simulink model "Tractor_HIT_Discrete"  (R2024a)
settings: Solver=ode1  StartTime=0.0  StopTime=60  FixedStep=0.001  RelTol=1e-3
values from neighbouring files (symbols this model uses):
  ANRtarget = 1.05    [Engine1204.sldd]    (also in Engine1204_init_r1.m; Engine2004.sldd; Engine2004_init.m; Engine3204.sldd)
  BackPrs = 3.0 4.2 5.5 7.0 8.5 10.0 11.5 12.5    [Engine1204.sldd]    (also in Engine1204_init_r1.m = [3.0, 4.2, 5.5, 7.0, 8.5, 10.0, 11.5, 12.5]; Engine2004.sldd = 3.0 4.2 5.5 7.0 8.5 10.0 11.5 12.5 13.5 14.5 15.0 15.5 16.0 ; Engine2004_init.m = [3.0,4.2,5.5,7.0,8.5,10.0,11.5,12.5,13.5,14.5,15.0,15.5,16.0; Engine3204.sldd = 3.0 4.5 6.0 7.5 9.0 10.5 12.0 13.0 13.8 14.4 14.8 15.2 15.6 )
  BackPrs_x = 50.0 100.0 150.0 200.0 250.0 300.0 350.0 400.0    [Engine1204.sldd]    (also in Engine1204_init_r1.m = [50:50:400]; Engine2004.sldd = 50.0 100.0 150.0 200.0 250.0 300.0 350.0 400.0 450.0 500.0 5; Engine2004_init.m = [50:50:800]; Engine3204.sldd = 100.0 200.0 300.0 400.0 500.0 600.0 700.0 800.0 900.0 1000.0)
  Bf = 0.38    [Engine1204.sldd]    (also in Engine2004.sldd; Engine3204.sldd)
  Br = 0.47    [Engine1204.sldd]    (also in Engine2004.sldd; Engine3204.sldd)
  BSFC = 320.0 285.0 275.0 280.0 290.0 300.0 310.0 260.0 225.0 215.0 220.0 228.0 240.0 250.0 235.0 208.0 202.0 205.0 212.0 222.0 232.0 230.0 205.0 200.0 204.0 210.0 220.0 230.0 232.0 207.0 203.0 206.0 213.0 224.0 235.0    [Engine1204.sldd]    (also in Engine1204_init_r1.m = [320,285,275,280,290,300,310; Engine2004.sldd = 315.0 280.0 270.0 275.0 285.0 295.0 305.0 255.0 220.0 210.0 ; Engine2004_init.m = [315,280,270,275,285,295,305; Engine3204.sldd = 310.0 275.0 265.0 270.0 280.0 290.0 300.0 250.0 215.0 205.0 )
  BSFC_x = 700.0 1200.0 1400.0 1600.0 1800.0 2000.0 2200.0    [Engine1204.sldd]    (also in Engine1204_init_r1.m = [700,1200,1400,1600,1800,2000,2200]; Engine2004.sldd = 800.0 1200.0 1400.0 1600.0 1800.0 2000.0 2200.0; Engine2004_init.m = [800,1200,1400,1600,1800,2000,2200]; Engine3204.sldd = 800.0 1000.0 1200.0 1400.0 1600.0 1800.0 2100.0)
  BSFC_y = 12.0 24.0 36.0 48.0 54.0    [Engine1204.sldd]    (also in Engine1204_init_r1.m = [12,24,36,48,54]; Engine2004.sldd = 20.0 40.0 60.0 80.0 100.0; Engine2004_init.m = [20,40,60,80,100]; Engine3204.sldd = 30.0 60.0 90.0 120.0 150.0)
  CO = 2.4 1.7 1.5 1.6 1.8 2.1 2.7 1.1 0.72 0.65 0.68 0.78 0.92 1.3 0.7 0.55 0.5 0.53 0.6 0.72 0.95 1.2 0.9 0.85 0.88 0.96 1.1 1.45 3.2 2.3 2.1 2.25 2.5 2.85 3.8    [Engine1204.sldd]    (also in Engine1204_init_r1.m = [; Engine2004.sldd = 2.3 1.63 1.44 1.54 1.73 2.02 2.56 1.05 0.68 0.61 0.64 0.74 0; Engine2004_init.m = [; Engine3204.sldd = 2.2 1.56 1.38 1.48 1.66 1.94 2.46 1.0 0.65 0.58 0.61 0.7 0.8)
  CO_x = 700.0 1200.0 1400.0 1600.0 1800.0 2000.0 2200.0    [Engine1204.sldd]    (also in Engine1204_init_r1.m = [700,1200,1400,1600,1800,2000,2200]; Engine2004.sldd = 800.0 1200.0 1400.0 1600.0 1800.0 2000.0 2200.0; Engine2004_init.m = [800,1200,1400,1600,1800,2000,2200]; Engine3204.sldd = 800.0 1000.0 1200.0 1400.0 1600.0 1800.0 2100.0)
  CO_y = 12.0 24.0 36.0 48.0 54.0    [Engine1204.sldd]    (also in Engine1204_init_r1.m = [12,24,36,48,54]; Engine2004.sldd = 20.0 40.0 60.0 80.0 100.0; Engine2004_init.m = [20,40,60,80,100]; Engine3204.sldd = 30.0 60.0 90.0 120.0 150.0)
  Df = 1.4    [Engine1204.sldd]    (also in Engine2004.sldd; Engine3204.sldd)
  dfmax = 0.1    [Engine1204.sldd]    (also in Engine2004.sldd; Engine3204.sldd)
  dfmin = 0.035    [Engine1204.sldd]    (also in Engine2004.sldd; Engine3204.sldd)
  DOCdPrs = 0.2 0.5 0.8 1.1 1.2    [Engine1204.sldd]    (also in Engine1204_init_r1.m = [0.2  0.5  0.8  1.1  1.2]; Engine2004.sldd = 0.25 0.55 0.85 1.15 1.3; Engine2004_init.m = [0.25,0.55,0.85,1.15,1.30]; Engine3204.sldd = 0.25 0.55 0.85 1.15 1.3 1.45)
  DOCdPrs_x = 50.0 150.0 250.0 350.0 400.0    [Engine1204.sldd]    (also in Engine1204_init_r1.m = [50  150  250  350  400]; Engine2004.sldd = 100.0 250.0 400.0 600.0 800.0; Engine2004_init.m = [100 250 400 600 800]; Engine3204.sldd = 100.0 250.0 400.0 600.0 800.0 1200.0)
  DPFdPrs = 0.3 0.5 0.7 0.9 0.6 1.0 1.4 1.8 0.9 1.5 2.1 2.6 1.2 2.0 2.7 2.8    [Engine1204.sldd]    (also in Engine1204_init_r1.m = [0.3  0.5  0.7  0.9; Engine2004.sldd = 0.35 0.6 0.85 1.1 0.7 1.15 1.6 2.0 1.05 1.7 2.3 2.5 1.4 2.2 ; Engine2004_init.m = [0.35,0.60,0.85,1.10; Engine3204.sldd = 0.35 0.7 1.05 1.4 1.7 2.0 2.2 2.4 2.55 2.65 2.7 2.75 0.6 1.1)
  DPFdPrs_x = 100.0 200.0 300.0 400.0    [Engine1204.sldd]    (also in Engine1204_init_r1.m = [100: 100 : 400]; Engine2004.sldd = 100.0 300.0 500.0 700.0; Engine2004_init.m = [100:200:700]; Engine3204.sldd = 100.0 200.0 300.0 400.0 500.0 600.0 700.0 800.0 900.0 1000.0)
  DPFdPrs_y = 0.0 6.0 12.0 20.0    [Engine1204.sldd]    (also in Engine1204_init_r1.m = [0 6 12 20 ]; Engine2004.sldd = 0.0 8.0 16.0 24.0; Engine2004_init.m = [0 8 16 24]; Engine3204.sldd = 0.0 10.0 20.0 30.0)
  DPFSootBurn = 0.0 0.0 0.0 0.0 0.0 0.2 0.4 0.6 0.8 1.0 1.2 2.4 3.6 4.8 6.0 6.0 12.0 18.0 24.0 30.0 12.0 24.0 36.0 48.0 60.0 20.0 40.0 60.0 80.0 100.0 22.0 44.0 66.0 88.0 110.0    [Engine1204.sldd]    (also in Engine1204_init_r1.m = [0,0,0,0,0; Engine2004.sldd = 0.0 0.0 0.0 0.0 0.0 0.5 1.0 1.5 2.0 2.5 3.0 6.0 9.0 12.0 15.; Engine2004_init.m = [0,0,0,0,0; Engine3204.sldd = 0.0 0.0 0.0 0.0 0.0 0.5 1.0 1.5 2.0 2.5 3.0 6.0 9.0 12.0 15.)
  DPFSootBurn_x = 100.0 200.0 300.0 400.0 500.0    [Engine1204.sldd]    (also in Engine1204_init_r1.m = [100,200,300,400,500]; Engine2004.sldd = 200.0 300.0 400.0 500.0 650.0; Engine2004_init.m = [200,300,400,500,650]; Engine3204.sldd = 200.0 300.0 400.0 500.0 650.0)
  DPFSootBurn_y = 400.0 450.0 500.0 550.0 600.0 650.0 680.0    [Engine1204.sldd]    (also in Engine1204_init_r1.m = [400,450,500,550,600,650,680]; Engine2004.sldd; Engine2004_init.m = [400,450,500,550,600,650,680]; Engine3204.sldd)
  Dr = 1.8    [Engine1204.sldd]    (also in Engine2004.sldd; Engine3204.sldd)
  drmax = 0.12    [Engine1204.sldd]    (also in Engine2004.sldd; Engine3204.sldd)
  drmin = 0.04    [Engine1204.sldd]    (also in Engine2004.sldd; Engine3204.sldd)
  EGRKi = 0.03    [Engine1204.sldd]    (also in Engine1204_init_r1.m; Engine2004.sldd; Engine2004_init.m; Engine3204.sldd)
  EGRKp = 3.5999999999999996    [Engine1204.sldd]    (also in Engine1204_init_r1.m = 3.6; Engine2004.sldd; Engine2004_init.m = 3.6; Engine3204.sldd)
  EGRMax = 1.0    [Engine1204.sldd]    (also in Engine1204_init_r1.m = 1; Engine2004.sldd; Engine2004_init.m = 1; Engine3204.sldd)
  EGRMin = 0.0    [Engine1204.sldd]    (also in Engine1204_init_r1.m = 0; Engine2004.sldd; Engine2004_init.m = 0; Engine3204.sldd)
  EGRRatio = 0.0 0.0 0.0 0.0 0.0 0.0 0.0 0.0 0.04 0.03 0.03 0.02 0.02 0.01 0.0 0.08 0.07 0.06 0.05 0.04 0.03 0.0 0.13 0.12 0.11 0.1 0.09 0.08 0.0 0.18 0.17 0.16 0.15 0.14 0.13 0.0 0.22 0.21 0.2 0.19 0.18 0.17    [Engine1204.sldd]    (also in Engine1204_init_r1.m = [; Engine2004.sldd; Engine2004_init.m = [; Engine3204.sldd)
  EGRRatio_x = 700.0 1200.0 1400.0 1600.0 1800.0 2000.0 2200.0    [Engine1204.sldd]    (also in Engine1204_init_r1.m = [700,1200,1400,1600,1800,2000,2200]; Engine2004.sldd = 800.0 1200.0 1400.0 1600.0 1800.0 2000.0 2200.0; Engine2004_init.m = [800,1200,1400,1600,1800,2000,2200]; Engine3204.sldd = 800.0 1000.0 1200.0 1400.0 1600.0 1800.0 2100.0)
  EGRRatio_y = 0.0 20.0 40.0 60.0 80.0 100.0    [Engine1204.sldd]    (also in Engine1204_init_r1.m = [0,20,40,60,80,100]; Engine2004.sldd; Engine2004_init.m = [0,20,40,60,80,100]; Engine3204.sldd)
  EGRTgt = 0.25 0.22 0.2 0.18 0.16 0.12 0.1 0.2 0.18 0.15 0.14 0.12 0.1 0.08 0.12 0.13 0.1 0.09 0.08 0.06 0.04 0.08 0.09 0.07 0.06 0.05 0.03 0.02 0.05 0.06 0.04 0.03 0.02 0.01 0.0    [Engine1204.sldd]    (also in Engine1204_init_r1.m = [0.25,0.22,0.20,0.18,0.16,0.12,0.10; Engine2004.sldd = 0.24 0.21 0.19 0.17 0.15 0.11 0.09 0.19 0.17 0.14 0.13 0.11 ; Engine2004_init.m = [0.24,0.21,0.19,0.17,0.15,0.11,0.09; Engine3204.sldd = 0.23 0.2 0.18 0.16 0.14 0.1 0.08 0.18 0.16 0.13 0.12 0.1 0.0)
  EGRTgt_x = 700.0 1200.0 1400.0 1600.0 1800.0 2000.0 2200.0    [Engine1204.sldd]    (also in Engine1204_init_r1.m = [700,1200,1400,1600,1800,2000,2200]; Engine2004.sldd = 800.0 1200.0 1400.0 1600.0 1800.0 2000.0 2200.0; Engine2004_init.m = [800,1200,1400,1600,1800,2000,2200]; Engine3204.sldd = 800.0 1000.0 1200.0 1400.0 1600.0 1800.0 2100.0)
  EGRTgt_y = 12.0 24.0 36.0 48.0 54.0    [Engine1204.sldd]    (also in Engine1204_init_r1.m = [12,24,36,48,54]; Engine2004.sldd = 20.0 40.0 60.0 80.0 100.0; Engine2004_init.m = [20,40,60,80,100]; Engine3204.sldd = 30.0 60.0 90.0 120.0 150.0)
  EGT = 197.0 257.0 287.0 297.0 287.0 267.0 247.0 267.0 357.0 397.0 407.0 392.0 367.0 347.0 337.0 437.0 472.0 482.0 462.0 437.0 407.0 367.0 477.0 502.0 512.0 492.0 467.0 437.0 377.0 487.0 510.0 520.0 500.0 477.0 447.0    [Engine1204.sldd]    (also in Engine1204_init_r1.m = [470,530,560,570,560,540,520; Engine2004.sldd = 187.0 247.0 277.0 287.0 277.0 257.0 237.0 257.0 347.0 387.0 ; Engine2004_init.m = [460,520,550,560,550,530,510; Engine3204.sldd = 307.0 327.0 338.0 327.0 307.0 277.0 237.0 322.0 337.0 332.0 )
  EGT_x = 700.0 1200.0 1400.0 1600.0 1800.0 2000.0 2200.0    [Engine1204.sldd]    (also in Engine1204_init_r1.m = [700,1200,1400,1600,1800,2000,2200]; Engine2004.sldd = 800.0 1200.0 1400.0 1600.0 1800.0 2000.0 2200.0; Engine2004_init.m = [800,1200,1400,1600,1800,2000,2200]; Engine3204.sldd = 800.0 1000.0 1200.0 1400.0 1600.0 1800.0 2100.0)
  EGT_y = 12.0 24.0 36.0 48.0 54.0    [Engine1204.sldd]    (also in Engine1204_init_r1.m = [12,24,36,48,54]; Engine2004.sldd = 20.0 40.0 60.0 80.0 100.0; Engine2004_init.m = [20,40,60,80,100]; Engine3204.sldd = 30.0 60.0 90.0 120.0 150.0)
  EngCsup = 0.35594 0.35501499999999997 0.353535 0.35242500000000004 0.351685 0.35150000000000003 0.35187 0.352795 0.35446 0.356865    [Engine1204.sldd]    (also in Engine2004.sldd; Engine3204.sldd)
  EngineSpdTgt = 700.0 850.0 1000.0 1150.0 1300.0 1450.0 1600.0 1750.0 1900.0 2050.0 2200.0    [Engine1204.sldd]    (also in Engine1204_init_r1.m = [700:150:2200]; Engine2004.sldd; Engine2004_init.m = [700:150:2200]; Engine3204.sldd = 800.0 930.0 1060.0 1190.0 1320.0 1450.0 1580.0 1710.0 1840.0)
  EngineSpdTgt_x = 0.0 10.0 20.0 30.0 40.0 50.0 60.0 70.0 80.0 90.0 100.0    [Engine1204.sldd]    (also in Engine1204_init_r1.m = [0:10:100]; Engine2004.sldd; Engine2004_init.m = [0:10:100]; Engine3204.sldd)
  EngineTrq = 70.0 110.0 130.0 125.0 115.0 100.0 85.0 180.0 280.0 320.0 310.0 285.0 250.0 220.0 260.0 370.0 410.0 395.0 365.0 320.0 280.0 300.0 420.0 450.0 435.0 400.0 350.0 300.0 310.0 435.0 460.0 445.0 410.0 355.0 305.0    [Engine1204.sldd]    (also in Engine1204_init_r1.m = [70,110,130,125,115,100,85; Engine2004.sldd = 130.0 200.0 240.0 230.0 210.0 180.0 150.0 320.0 480.0 550.0 ; Engine2004_init.m = [130,200,240,230,210,180,150; Engine3204.sldd = 210.0 320.0 380.0 360.0 330.0 290.0 240.0 510.0 760.0 870.0 )
  EngineTrq_x = 700.0 1200.0 1400.0 1600.0 1800.0 2000.0 2200.0    [Engine1204.sldd]    (also in Engine1204_init_r1.m = [700,1200,1400,1600,1800,2000,2200]; Engine2004.sldd = 800.0 1200.0 1400.0 1600.0 1800.0 2000.0 2200.0; Engine2004_init.m = [800,1200,1400,1600,1800,2000,2200]; Engine3204.sldd = 800.0 1000.0 1200.0 1400.0 1600.0 1800.0 2100.0)
  EngineTrq_y = 12.0 24.0 36.0 48.0 54.0    [Engine1204.sldd]    (also in Engine1204_init_r1.m = [12,24,36,48,54]; Engine2004.sldd = 20.0 40.0 60.0 80.0 100.0; Engine2004_init.m = [20,40,60,80,100]; Engine3204.sldd = 30.0 60.0 90.0 120.0 150.0)
  EngSpd = 800.0 1000.0 1200.0 1400.0 1600.0 1800.0 2000.0 2200.0 2400.0 2600.0    [Engine1204.sldd]    (also in Engine2004.sldd; Engine3204.sldd)
  EngTrq = 667.0 700.0 768.0 830.0 885.0 860.0 789.0 690.0 542.0 352.0    [Engine1204.sldd]    (also in Engine2004.sldd; Engine3204.sldd)
  etaCO = 0.0 0.0 0.0 0.0 0.6 0.45 0.3 0.15 0.92 0.85 0.75 0.6 0.98 0.95 0.9 0.82 0.99 0.97 0.94 0.88    [Engine1204.sldd]    (also in Engine1204_init_r1.m = [0.00	0.00	0.00	0.00; Engine2004.sldd; Engine2004_init.m = [0.00	0.00	0.00	0.00; Engine3204.sldd)
  etaCO_x = 10000.0 25000.0 40000.0 60000.0    [Engine1204.sldd]    (also in Engine1204_init_r1.m = [10000  25000  40000  60000]; Engine2004.sldd; Engine2004_init.m = [10000 25000 40000 60000]; Engine3204.sldd)
  etaCO_y = 120.0 200.0 280.0 360.0 450.0    [Engine1204.sldd]    (also in Engine1204_init_r1.m = [120, 200, 280, 360, 450]; Engine2004.sldd; Engine2004_init.m = [120,200,280,360,450]; Engine3204.sldd)
  etaHC = 0.0 0.0 0.0 0.0 0.5 0.35 0.2 0.1 0.88 0.8 0.68 0.5 0.96 0.92 0.86 0.75 0.98 0.95 0.91 0.83    [Engine1204.sldd]    (also in Engine1204_init_r1.m = [0.00	0.00	0.00	0.00; Engine2004.sldd; Engine2004_init.m = [0.00	0.00	0.00	0.00; Engine3204.sldd)
  etaHC_x = 10000.0 25000.0 40000.0 60000.0    [Engine1204.sldd]    (also in Engine1204_init_r1.m = [10000  25000  40000  60000]; Engine2004.sldd; Engine2004_init.m = [10000 25000 40000 60000]; Engine3204.sldd)
  etaHC_y = 120.0 200.0 280.0 360.0 450.0    [Engine1204.sldd]    (also in Engine1204_init_r1.m = [120, 200, 280, 360, 450]; Engine2004.sldd; Engine2004_init.m = [120,200,280,360,450]; Engine3204.sldd)
  etaNO2 = 0.0 0.0 0.0 0.0 0.2 0.15 0.1 0.05 0.4 0.33 0.25 0.18 0.55 0.48 0.4 0.3 0.6 0.53 0.45 0.35    [Engine1204.sldd]    (also in Engine1204_init_r1.m = [0.00	0.00	0.00	0.00; Engine2004.sldd; Engine2004_init.m = [0.00	0.00	0.00	0.00; Engine3204.sldd)
  etaNO2_x = 10000.0 25000.0 40000.0 60000.0    [Engine1204.sldd]    (also in Engine1204_init_r1.m = [10000  25000  40000  60000]; Engine2004.sldd; Engine2004_init.m = [10000 25000 40000 60000]; Engine3204.sldd)
  etaNO2_y = 120.0 200.0 280.0 360.0 450.0    [Engine1204.sldd]    (also in Engine1204_init_r1.m = [120, 200, 280, 360, 450]; Engine2004.sldd; Engine2004_init.m = [120,200,280,360,450]; Engine3204.sldd)
  etaPM = 0.995 0.992 0.988 0.98 0.996 0.994 0.99 0.985 0.997 0.995 0.992 0.988    [Engine1204.sldd]    (also in Engine1204_init_r1.m = [0.995  0.992  0.988  0.980; Engine2004.sldd; Engine2004_init.m = [0.995  0.992  0.988  0.980; Engine3204.sldd)
  etaPM_x = 10000.0 25000.0 40000.0 60000.0    [Engine1204.sldd]    (also in Engine1204_init_r1.m = [10000  25000  40000  60000]; Engine2004.sldd; Engine2004_init.m = [10000 25000 40000 60000]; Engine3204.sldd)
  etaPM_y = 150.0 300.0 450.0    [Engine1204.sldd]    (also in Engine1204_init_r1.m = [150, 300, 450]; Engine2004.sldd; Engine2004_init.m = [150,300,450]; Engine3204.sldd)
  FuelCyleMax = 40.0 45.0 50.0 52.0 54.0 50.0 60.0 65.0 66.0 68.0 52.0 64.0 66.0 67.0 68.0 50.0 62.0 64.0 65.0 66.0 48.0 58.0 60.0 61.0 62.0 42.0 50.0 52.0 53.0 54.0 38.0 44.0 46.0 47.0 48.0    [Engine1204.sldd]    (also in Engine1204_init_r1.m = [40,45,50,52,54; Engine2004.sldd = 65.0 75.0 82.0 88.0 92.0 75.0 88.0 94.0 98.0 102.0 78.0 92.0; Engine2004_init.m = [65,75,82,88,92; Engine3204.sldd = 95.0 110.0 125.0 140.0 155.0 110.0 130.0 145.0 160.0 175.0 1)
  FuelCyleMax_x = 80.0 140.0 200.0 260.0 320.0    [Engine1204.sldd]    (also in Engine1204_init_r1.m = [80,140,200,260,320]; Engine2004.sldd = 150.0 300.0 450.0 600.0 750.0; Engine2004_init.m = [150,300,450,600,750]; Engine3204.sldd = 250.0 500.0 750.0 1000.0 1300.0)
  FuelCyleMax_y = 700.0 1200.0 1400.0 1600.0 1800.0 2000.0 2200.0    [Engine1204.sldd]    (also in Engine1204_init_r1.m = [700,1200,1400,1600,1800,2000,2200]; Engine2004.sldd = 800.0 1200.0 1400.0 1600.0 1800.0 2000.0 2200.0; Engine2004_init.m = [800,1200,1400,1600,1800,2000,2200]; Engine3204.sldd = 800.0 1000.0 1200.0 1400.0 1600.0 1800.0 2100.0)
  FuelCyleMaxSw = 0.0    [Engine1204.sldd]    (also in Engine1204_init_r1.m = 0; Engine2004.sldd; Engine2004_init.m = 0; Engine3204.sldd)
  FuelCyleMin = 10.0    [Engine1204.sldd]    (also in Engine1204_init_r1.m = 10; Engine2004.sldd = 12.0; Engine2004_init.m = 12; Engine3204.sldd = 15.0)
  FuelKd = 0.0    [Engine1204.sldd]    (also in Engine1204_init_r1.m = 0; Engine2004.sldd; Engine2004_init.m = 0; Engine3204.sldd)
  FuelKi = 0.0162    [Engine1204.sldd]    (also in Engine1204_init_r1.m; Engine2004.sldd = 0.0198; Engine2004_init.m = 0.0198; Engine3204.sldd = 0.025199999999999997)
  FuelKp = 0.054    [Engine1204.sldd]    (also in Engine1204_init_r1.m; Engine2004.sldd = 0.066; Engine2004_init.m = 0.066; Engine3204.sldd = 0.083999999999999991)
  g = 9.81    [Engine1204.sldd]    (also in Engine2004.sldd; Engine3204.sldd)
  GearA = -2.9 0.0 6.0 2.5 1.0    [Engine1204.sldd]    (also in Engine2004.sldd; Engine3204.sldd)
  GearAC = -1.0 0.0 1.0 2.0 3.0    [Engine1204.sldd]    (also in Engine2004.sldd; Engine3204.sldd)
  GearFront = 17.574    [Engine1204.sldd]    (also in Engine2004.sldd; Engine3204.sldd)
  GearM = 2.33 1.75 1.4 1.0    [Engine1204.sldd]    (also in Engine2004.sldd; Engine3204.sldd)
  GearMC = 1.0 2.0 3.0 4.0    [Engine1204.sldd]    (also in Engine2004.sldd; Engine3204.sldd)
  GearRef = 14.6    [Engine1204.sldd]    (also in Engine2004.sldd; Engine3204.sldd)
  HC = 0.85 0.6 0.52 0.55 0.62 0.7 0.9 0.4 0.22 0.2 0.21 0.26 0.32 0.48 0.25 0.18 0.17 0.18 0.21 0.26 0.36 0.32 0.24 0.23 0.25 0.28 0.33 0.42 0.55 0.42 0.4 0.43 0.48 0.54 0.68    [Engine1204.sldd]    (also in Engine1204_init_r1.m = [; Engine2004.sldd = 0.82 0.58 0.5 0.53 0.6 0.68 0.87 0.38 0.21 0.19 0.2 0.24 0.3; Engine2004_init.m = [; Engine3204.sldd = 0.8 0.56 0.48 0.51 0.58 0.66 0.84 0.37 0.2 0.18 0.19 0.23 0.)
  HC_x = 700.0 1200.0 1400.0 1600.0 1800.0 2000.0 2200.0    [Engine1204.sldd]    (also in Engine1204_init_r1.m = [700,1200,1400,1600,1800,2000,2200]; Engine2004.sldd = 800.0 1200.0 1400.0 1600.0 1800.0 2000.0 2200.0; Engine2004_init.m = [800,1200,1400,1600,1800,2000,2200]; Engine3204.sldd = 800.0 1000.0 1200.0 1400.0 1600.0 1800.0 2100.0)
  HC_y = 12.0 24.0 36.0 48.0 54.0    [Engine1204.sldd]    (also in Engine1204_init_r1.m = [12,24,36,48,54]; Engine2004.sldd = 20.0 40.0 60.0 80.0 100.0; Engine2004_init.m = [20,40,60,80,100]; Engine3204.sldd = 30.0 60.0 90.0 120.0 150.0)
  hf = 0.35    [Engine1204.sldd]    (also in Engine2004.sldd; Engine3204.sldd)
  hr = 0.4    [Engine1204.sldd]    (also in Engine2004.sldd; Engine3204.sldd)
  IdleEngSpd = 700.0    [Engine1204.sldd]    (also in Engine2004.sldd; Engine3204.sldd)
  IdleThrottle = 0.3    [Engine1204.sldd]    (also in Engine2004.sldd; Engine3204.sldd)
  Inertia = 0.9    [Engine1204.sldd]    (also in Engine1204_init_r1.m; Engine2004.sldd = 1.4; Engine2004_init.m = 1.4; Engine3204.sldd = 2.0)
  Intake = 80.0 140.0 160.0 180.0 190.0 195.0 200.0 130.0 210.0 240.0 260.0 270.0 275.0 280.0 170.0 270.0 310.0 330.0 340.0 345.0 350.0 190.0 320.0 360.0 380.0 390.0 395.0 400.0 200.0 340.0 380.0 400.0 410.0 415.0 420.0    [Engine1204.sldd]    (also in Engine1204_init_r1.m = [80,140,160,180,190,195,200; Engine2004.sldd = 160.0 240.0 280.0 310.0 330.0 340.0 350.0 250.0 380.0 440.0 ; Engine2004_init.m = [160,240,280,310,330,340,350; Engine3204.sldd = 280.0 420.0 490.0 540.0 570.0 585.0 600.0 430.0 660.0 760.0 )
  Intake_x = 700.0 1200.0 1400.0 1600.0 1800.0 2000.0 2200.0    [Engine1204.sldd]    (also in Engine1204_init_r1.m = [700,1200,1400,1600,1800,2000,2200]; Engine2004.sldd = 800.0 1200.0 1400.0 1600.0 1800.0 2000.0 2200.0; Engine2004_init.m = [800,1200,1400,1600,1800,2000,2200]; Engine3204.sldd = 800.0 1000.0 1200.0 1400.0 1600.0 1800.0 2100.0)
  Intake_y = 12.0 24.0 36.0 48.0 54.0    [Engine1204.sldd]    (also in Engine1204_init_r1.m = [12,24,36,48,54]; Engine2004.sldd = 20.0 40.0 60.0 80.0 100.0; Engine2004_init.m = [20,40,60,80,100]; Engine3204.sldd = 30.0 60.0 90.0 120.0 150.0)
  IntakePrs = 1.0 1.1 1.22 1.35 1.48 1.6 1.7 1.0 1.12 1.24 1.37 1.5 1.62 1.72 1.0 1.13 1.25 1.38 1.51 1.63 1.73 1.0 1.14 1.26 1.39 1.52 1.64 1.74 1.0 1.15 1.27 1.4 1.53 1.65 1.75 1.0 1.16 1.28 1.41 1.54 1.66 1.76    [Engine1204.sldd]    (also in Engine1204_init_r1.m = [; Engine2004.sldd = 1.0 1.11 1.23 1.36 1.49 1.61 1.71 1.0 1.13 1.25 1.38 1.51 1.; Engine2004_init.m = [; Engine3204.sldd = 1.0 1.12 1.24 1.37 1.5 1.62 1.72 1.0 1.14 1.26 1.39 1.52 1.6)
  IntakePrs_x = 700.0 1200.0 1400.0 1600.0 1800.0 2000.0 2200.0    [Engine1204.sldd]    (also in Engine1204_init_r1.m = [700,1200,1400,1600,1800,2000,2200]; Engine2004.sldd = 800.0 1200.0 1400.0 1600.0 1800.0 2000.0 2200.0; Engine2004_init.m = [800,1200,1400,1600,1800,2000,2200]; Engine3204.sldd = 800.0 1000.0 1200.0 1400.0 1600.0 1800.0 2100.0)
  IntakePrs_y = 0.0 20.0 40.0 60.0 80.0 100.0    [Engine1204.sldd]    (also in Engine1204_init_r1.m = [0,20,40,60,80,100]; Engine2004.sldd; Engine2004_init.m = [0,20,40,60,80,100]; Engine3204.sldd)
  IntakePrsInit = 1.35    [Engine1204.sldd]    (also in Engine1204_init_r1.m; Engine2004.sldd; Engine2004_init.m; Engine3204.sldd)
  IntakeSw = 0    [Engine1204.sldd]    (also in Engine1204_init_r1.m = false; Engine2004.sldd; Engine2004_init.m = false; Engine3204.sldd)
  IntakeTC = 0.1    [Engine1204.sldd]    (also in Engine1204_init_r1.m; Engine2004.sldd; Engine2004_init.m; Engine3204.sldd)
  IntakeTemp = 25.0 28.0 30.0 32.0 34.0 36.0 38.0 25.0 38.0 40.0 42.0 44.0 46.0 48.0 25.0 48.0 50.0 52.0 54.0 56.0 58.0 25.0 58.0 60.0 62.0 64.0 66.0 68.0 25.0 66.0 68.0 70.0 72.0 74.0 76.0 25.0 72.0 74.0 76.0 78.0 80.0 82.0    [Engine1204.sldd]    (also in Engine1204_init_r1.m = [; Engine2004.sldd = 25.0 29.0 31.0 33.0 35.0 37.0 39.0 25.0 39.0 41.0 43.0 45.0 ; Engine2004_init.m = [; Engine3204.sldd = 25.0 30.0 32.0 34.0 36.0 38.0 40.0 25.0 40.0 42.0 44.0 46.0 )
  IntakeTemp_x = 700.0 1200.0 1400.0 1600.0 1800.0 2000.0 2200.0    [Engine1204.sldd]    (also in Engine1204_init_r1.m = [700,1200,1400,1600,1800,2000,2200]; Engine2004.sldd = 800.0 1200.0 1400.0 1600.0 1800.0 2000.0 2200.0; Engine2004_init.m = [800,1200,1400,1600,1800,2000,2200]; Engine3204.sldd = 800.0 1000.0 1200.0 1400.0 1600.0 1800.0 2100.0)
  IntakeTemp_y = 0.0 20.0 40.0 60.0 80.0 100.0    [Engine1204.sldd]    (also in Engine1204_init_r1.m = [0,20,40,60,80,100]; Engine2004.sldd; Engine2004_init.m = [0,20,40,60,80,100]; Engine3204.sldd)
  IntakeTempInit = 45.0    [Engine1204.sldd]    (also in Engine1204_init_r1.m = 45; Engine2004.sldd; Engine2004_init.m = 45; Engine3204.sldd)
  Jf = 180.0    [Engine1204.sldd]    (also in Engine2004.sldd; Engine3204.sldd)
  Jr = 450.0    [Engine1204.sldd]    (also in Engine2004.sldd; Engine3204.sldd)
  L = 2.75    [Engine1204.sldd]    (also in Engine2004.sldd; Engine3204.sldd)
  LiftTorque = 5000.0    [Engine1204.sldd]    (also in Engine2004.sldd; Engine3204.sldd)
  LoadTrqManu = 200.0    [Engine1204.sldd]    (also in Engine1204_init_r1.m = 200; Engine2004.sldd = 400.0; Engine2004_init.m = 400; Engine3204.sldd = 800.0)
  LoadTrqSW = 1    [Engine1204.sldd]    (also in Engine1204_init_r1.m = true; Engine2004.sldd; Engine2004_init.m = true; Engine3204.sldd = 0)
  M_I = 2500.0    [Engine1204.sldd]    (also in Engine2004.sldd; Engine3204.sldd)
  M_T = 6500.0    [Engine1204.sldd]    (also in Engine2004.sldd; Engine3204.sldd)
  MaxEngSpd = 2600.0    [Engine1204.sldd]    (also in Engine2004.sldd; Engine3204.sldd)
  NH3StoreMax = 0.0 1.2 2.0 2.4 2.2 1.7 1.1    [Engine1204.sldd]    (also in Engine1204_init_r1.m = [0  1.2  2.0  2.4  2.2  1.7  1.1]; Engine2004.sldd = 0.0 1.7 2.9 3.5 3.2 2.5 1.6; Engine2004_init.m = [0, 1.7, 2.9, 3.5, 3.2, 2.5, 1.6]; Engine3204.sldd = 0.0 2.2 3.8 4.5 4.2 3.3 2.1)
  NH3StoreMax_x = 180.0 220.0 260.0 300.0 340.0 380.0 420.0    [Engine1204.sldd]    (also in Engine1204_init_r1.m = [180  220  260  300  340  380  420]; Engine2004.sldd; Engine2004_init.m = [180 220 260 300 340 380 420]; Engine3204.sldd)
  NOx = 6.2 7.0 7.4 7.2 6.8 6.4 6.0 7.5 8.4 8.8 8.6 8.2 7.7 7.2 8.2 9.1 9.5 9.3 8.9 8.4 7.9 7.6 8.5 8.8 8.6 8.2 7.7 7.2 7.0 7.8 8.1 7.9 7.5 7.0 6.5    [Engine1204.sldd]    (also in Engine1204_init_r1.m = [6.2,7.0,7.4,7.2,6.8,6.4,6.0; Engine2004.sldd = 6.1 6.9 7.3 7.1 6.7 6.3 5.9 7.4 8.3 8.7 8.5 8.1 7.6 7.1 8.1 ; Engine2004_init.m = [6.1,6.9,7.3,7.1,6.7,6.3,5.9; Engine3204.sldd = 5.9 6.7 7.1 6.9 6.5 6.1 5.7 7.2 8.1 8.5 8.3 7.9 7.4 6.9 7.9 )
  NOx_x = 700.0 1200.0 1400.0 1600.0 1800.0 2000.0 2200.0    [Engine1204.sldd]    (also in Engine1204_init_r1.m = [700,1200,1400,1600,1800,2000,2200]; Engine2004.sldd = 800.0 1200.0 1400.0 1600.0 1800.0 2000.0 2200.0; Engine2004_init.m = [800,1200,1400,1600,1800,2000,2200]; Engine3204.sldd = 800.0 1000.0 1200.0 1400.0 1600.0 1800.0 2100.0)
  NOx_y = 12.0 24.0 36.0 48.0 54.0    [Engine1204.sldd]    (also in Engine1204_init_r1.m = [12,24,36,48,54]; Engine2004.sldd = 20.0 40.0 60.0 80.0 100.0; Engine2004_init.m = [20,40,60,80,100]; Engine3204.sldd = 30.0 60.0 90.0 120.0 150.0)
  NOxFac = 1.0 0.88 0.76 0.64 0.54 0.46 0.4    [Engine1204.sldd]    (also in Engine1204_init_r1.m = [1.00, 0.88, 0.76, 0.64, 0.54, 0.46, 0.40]; Engine2004.sldd; Engine2004_init.m = [1.00,0.88,0.76,0.64,0.54,0.46,0.40]; Engine3204.sldd)
  NOxFac_x = 0.0 0.05 0.1 0.15 0.19999999999999998 0.25 0.3    [Engine1204.sldd]    (also in Engine1204_init_r1.m = [0: 0.05 : 0.3]; Engine2004.sldd; Engine2004_init.m = [0:0.05:0.3]; Engine3204.sldd)
  NumCyl = 6.0    [Engine1204.sldd]    (also in Engine1204_init_r1.m = 6; Engine2004.sldd; Engine2004_init.m = 6; Engine3204.sldd)
  O2 = 16.5 16.0 15.8 15.5 15.2 14.8 14.5 13.0 12.2 11.8 11.5 11.2 10.8 10.5 9.5 8.6 8.0 7.7 7.4 7.0 6.7 7.0 6.2 5.6 5.3 5.0 4.7 4.4 6.0 5.3 4.8 4.5 4.2 4.0 3.8    [Engine1204.sldd]    (also in Engine1204_init_r1.m = [16.5,16.0,15.8,15.5,15.2,14.8,14.5; Engine2004.sldd = 16.3 15.8 15.6 15.3 15.0 14.6 14.3 12.8 12.0 11.6 11.3 11.0 ; Engine2004_init.m = [16.3,15.8,15.6,15.3,15.0,14.6,14.3; Engine3204.sldd = 16.0 15.5 15.3 15.0 14.7 14.3 14.0 12.5 11.7 11.3 11.0 10.7 )
  O2_x = 700.0 1200.0 1400.0 1600.0 1800.0 2000.0 2200.0    [Engine1204.sldd]    (also in Engine1204_init_r1.m = [700,1200,1400,1600,1800,2000,2200]; Engine2004.sldd = 800.0 1200.0 1400.0 1600.0 1800.0 2000.0 2200.0; Engine2004_init.m = [800,1200,1400,1600,1800,2000,2200]; Engine3204.sldd = 800.0 1000.0 1200.0 1400.0 1600.0 1800.0 2100.0)
  O2_y = 12.0 24.0 36.0 48.0 54.0    [Engine1204.sldd]    (also in Engine1204_init_r1.m = [12,24,36,48,54]; Engine2004.sldd = 20.0 40.0 60.0 80.0 100.0; Engine2004_init.m = [20,40,60,80,100]; Engine3204.sldd = 30.0 60.0 90.0 120.0 150.0)
  PM = 0.12 0.1 0.09 0.09 0.1 0.11 0.12 0.22 0.18 0.16 0.17 0.19 0.21 0.24 0.38 0.3 0.26 0.27 0.31 0.35 0.39 0.55 0.44 0.38 0.4 0.45 0.5 0.56 0.65 0.52 0.46 0.48 0.53 0.58 0.66    [Engine1204.sldd]    (also in Engine1204_init_r1.m = [0.12,0.10,0.09,0.09,0.10,0.11,0.12; Engine2004.sldd = 0.11 0.09 0.08 0.08 0.09 0.1 0.11 0.21 0.17 0.15 0.16 0.18 0; Engine2004_init.m = [0.11,0.09,0.08,0.08,0.09,0.10,0.11; Engine3204.sldd = 0.1 0.08 0.07 0.07 0.08 0.09 0.1 0.2 0.16 0.14 0.15 0.17 0.1)
  PM_x = 700.0 1200.0 1400.0 1600.0 1800.0 2000.0 2200.0    [Engine1204.sldd]    (also in Engine1204_init_r1.m = [700,1200,1400,1600,1800,2000,2200]; Engine2004.sldd = 800.0 1200.0 1400.0 1600.0 1800.0 2000.0 2200.0; Engine2004_init.m = [800,1200,1400,1600,1800,2000,2200]; Engine3204.sldd = 800.0 1000.0 1200.0 1400.0 1600.0 1800.0 2100.0)
  PM_y = 12.0 24.0 36.0 48.0 54.0    [Engine1204.sldd]    (also in Engine1204_init_r1.m = [12,24,36,48,54]; Engine2004.sldd = 20.0 40.0 60.0 80.0 100.0; Engine2004_init.m = [20,40,60,80,100]; Engine3204.sldd = 30.0 60.0 90.0 120.0 150.0)
  radps2rpm = 9.55    [Engine1204.sldd]    (also in Engine1204_init_r1.m; Engine2004.sldd; Engine2004_init.m; Engine3204.sldd)
  RailFuel = 400.0 600.0 700.0 700.0 650.0 600.0 550.0 600.0 800.0 900.0 900.0 850.0 800.0 750.0 700.0 1000.0 1100.0 1150.0 1100.0 1000.0 950.0 750.0 1200.0 1350.0 1350.0 1300.0 1200.0 1150.0 750.0 1300.0 1400.0 1450.0 1400.0 1300.0 1200.0    [Engine1204.sldd]    (also in Engine1204_init_r1.m = [400,600,700,700,650,600,550; Engine2004.sldd = 420.0 620.0 720.0 720.0 680.0 630.0 580.0 630.0 830.0 930.0 ; Engine2004_init.m = [420,620,720,720,680,630,580; Engine3204.sldd = 440.0 640.0 740.0 740.0 700.0 650.0 600.0 650.0 850.0 950.0 )
  RailFuel_x = 700.0 1200.0 1400.0 1600.0 1800.0 2000.0 2200.0    [Engine1204.sldd]    (also in Engine1204_init_r1.m = [700,1200,1400,1600,1800,2000,2200]; Engine2004.sldd = 800.0 1200.0 1400.0 1600.0 1800.0 2000.0 2200.0; Engine2004_init.m = [800,1200,1400,1600,1800,2000,2200]; Engine3204.sldd = 800.0 1000.0 1200.0 1400.0 1600.0 1800.0 2100.0)
  ... (+23 more)
undefined symbols (not defined in the file or in its folder): df, DiscIntNeverNeededParam, dr, MAP_AIR, MAP_EFF, MAP_EoCO, MAP_EoCO2, MAP_EoHC, MAP_EoNOx, MAP_EoPM, MAP_FUEL, MAP_FUELCMD, MAP_POWER, MAP_SPD, MAP_TEMPERATURE, NH3_MAX, R
libraries: simulink x9, slpidlib x5
(part 1 of 10)
settings Model: Creator=qixin.yang  LastModifiedBy=jhh
settings SolverCC: AlgebraicLoopSolver=TrustRegion
settings OptimizationCC: ReuseModelBlockBuffer=off
settings DebuggingCC: UnconnectedInputMsg=warning  UnconnectedOutputMsg=warning  UnconnectedLineMsg=warning  ArithmeticOperatorsInVariantConditions=warning
settings ModelReferenceCC: EnableRefExpFcnMdlSchedulingChecks=on
settings SFSimCC: CustomCodeUndefinedFunction=UseInterfaceOnly
settings RTWCC: GPUComputeCapability=3.5

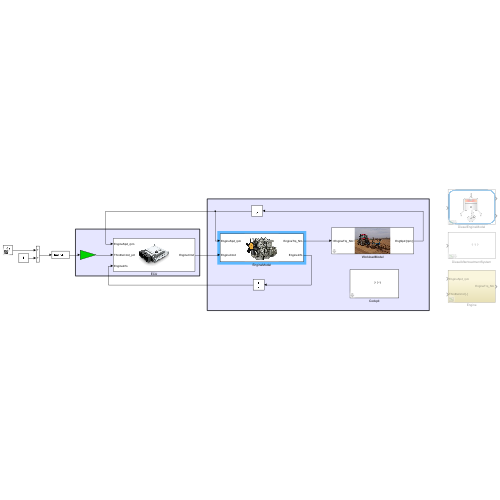
[thumbnail: Simulink's stored preview of the top-level diagram]
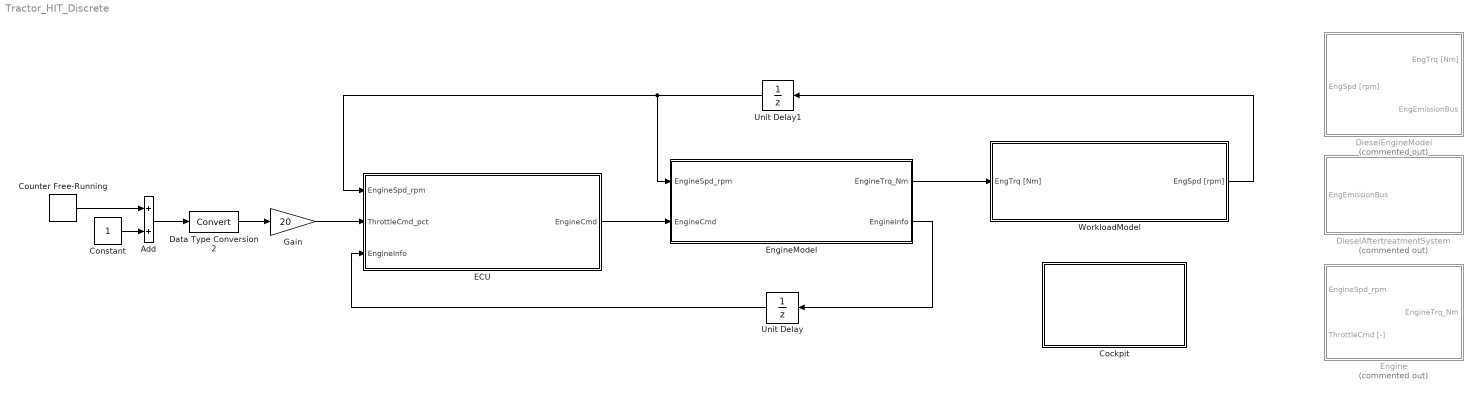
== system Tractor_HIT_Discrete ==
  Add : Sum
  Cockpit : Subsystem  mask{FSCmd=1, GearMCmd=3, GearACmd=2, DriveCmd=1, ThrottleCmd=50, Scene=1, Soil=1, Moisture=10, Density=1.6, Terrain=0, TypeCmd=1, PTOSpdCmd=1, TravelDistance=200}
      mask prompts: FSCmd "慢快档 0-Slow，1-Fast"; GearMCmd "主变速器 0 1 2 3"; GearACmd "辅变速器 0-R 1-N 2-L 3-M 4-H"; DriveCmd "驱动模式 0-Rear,1-Four"; ThrottleCmd "油门(%)"; Scene "场景 0-水田,1-旱田,2-果园"; Soil "土质 0-粘土, 1-壤土, 2-砂土"; Moisture "土壤含水量(%)"; Density "土壤容重(g/cm3)"; Terrain "地形 0-平坦 1-起伏 2-陡峭"; TypeCmd "农机类型 0-耕耘机 1-铧式犁 2-扫地犁 3-深松机 4-凿式犁 5-水田犁 6-PTO"; PTOSpdCmd "PTO 0-无需求 1-540rpm 2-1000rpm 3-同步转速"; TravelDistance "掉头距离(m)"
      mask DialogControl ParameterGroupVar Prompt: 参数
      mask Display: image('cockpit.png'); % 使用工具条上的 "编辑图像" 进行更改。
  Constant : Constant
  Counter Free-Running : simulink/Sources/Counter Free-Running  NumBits=2  tsamp=20
  Data Type Conversion2 : DataTypeConversion  SaturateOnIntegerOverflow=off  RndMeth=Floor
  DieselAftertreatmentSystem : Subsystem  Commented=on  mask{Parameter1=0}
      mask Display: image('after.png'); % 使用工具条上的 "编辑图像" 进行更改。
  DieselEngineModel : Subsystem  Commented=on  mask{Parameter1=0}
      mask Display: image('engine.png'); % 使用工具条上的 "编辑图像" 进行更改。
  ECU : Subsystem
      mask Display: image('ECU.jpeg', [30,10,30,10,100,100]);
  Engine : Subsystem  Commented=on
  EngineModel : Subsystem
      mask Display: image('Engine.jpg', [30,0,30,0,100,100]);
  Gain : Gain  Gain=20
  Unit Delay : UnitDelay  SampleTime=-1  HasFrameUpgradeWarning=on
  Unit Delay1 : UnitDelay  SampleTime=-1  HasFrameUpgradeWarning=on
  WorkloadModel : Subsystem  mask{Parameter1=0}
      mask DialogControl ParameterGroupVar Prompt: 参数
      mask Display: image('Tractor.jpg', [30,0,30,0,100,100]);
  wires:
  Data Type Conversion2/1 -> Gain/1
  Gain/1 -> ECU/2(ThrottleCmd_pct)
  Add/1 -> Data Type Conversion2/1
  Counter Free-Running/1 -> Add/1
  Constant/1 -> Add/2
  Unit Delay/1 -> ECU/3(EngineInfo)
  EngineModel/2(EngineInfo) -> Unit Delay/1
  ECU/1(EngineCmd) -> EngineModel/2(EngineCmd)
  Unit Delay1/1 -> ECU/1(EngineSpd_rpm), EngineModel/1(EngineSpd_rpm)
  EngineModel/1(EngineTrq_Nm) -> WorkloadModel/1(EngTrq [Nm])
  WorkloadModel/1(EngSpd [rpm]) -> Unit Delay1/1

== system Tractor_HIT_Discrete/Cockpit ==
  note: Driver
  Bias : Bias  Bias=1  SaturateOnIntegerOverflow=off
  Bias1 : Bias  Bias=-1  SaturateOnIntegerOverflow=off
  Bus Creator : BusCreator  Inputs=3
  Bus Creator2 : BusCreator  Inputs=4
  Density [g/cm3] : Constant  Value=Density
  DriveCmd [-] : Constant  Value=DriveCmd
  FastSlowCmd [-] : Constant  Value=FSCmd
  Gain1 : Gain  Gain=0.01
  GearACmd [-] : Constant  Value=GearACmd
  GearMCmd [-] : Constant  Value=GearMCmd
  Moisture [%] : Constant  Value=Moisture
  PTOSpdCmd [-] : Constant  Value=PTOSpdCmd
  Scene : Constant  Value=Scene
  Soil [-] : Constant  Value=Soil
  Terrain [-] : Constant  Value=Terrain
  ThrottleCmd [%] : Constant  Value=ThrottleCmd
  TravelDistance[m] : Constant  Value=TravelDistance
  TypeCmd [-] : Constant  Value=TypeCmd
  tag scope: DriveCmd=global, GearCmd=global, Land=global, PTOSpdCmd=global, Scene=global, ThrottleCmd=global, TravelDistance=global, TypeCmd=global
  wires:
  Terrain [-]/1 -> Bus Creator2/4  "Terrain"
  Bias/1 -> Bus Creator/2  "GearMCmd"
  FastSlowCmd [-]/1 -> Bus Creator/1  "FastSlowCmd"
  Gain1/1 -> [ThrottleCmd]
  DriveCmd [-]/1 -> [DriveCmd]
  ThrottleCmd [%]/1 -> Gain1/1
  TypeCmd [-]/1 -> [TypeCmd]
  TravelDistance[m]/1 -> [TravelDistance]
  Scene/1 -> [Scene]
  Bias1/1 -> Bus Creator/3  "GearACmd"
  Density [g/cm3]/1 -> Bus Creator2/3  "Density"
  Bus Creator/1 -> [GearCmd]
  GearMCmd [-]/1 -> Bias/1
  Moisture [%]/1 -> Bus Creator2/2  "Moisture"
  Bus Creator2/1 -> [Land]
  Soil [-]/1 -> Bus Creator2/1  "Soil"
  PTOSpdCmd [-]/1 -> [PTOSpdCmd]
  GearACmd [-]/1 -> Bias1/1

== system Tractor_HIT_Discrete/DieselAftertreatmentSystem ==
  EngEmissionBus : Inport
  Bus Selector : BusSelector  OutputSignals=EngFuel[mL/s],EngPwr[kW]
  DOC : Subsystem
  DPF : Subsystem
  Gain : Gain  Gain=3.6
  Gain2 : Gain  Gain=3.6
  Mux : Mux  Inputs=3
  SCR : Subsystem
  Scope1 : Scope  NumInputPorts=4
  Scope2 : Scope  NumInputPorts=3
  Statistics : Subsystem
  tag scope: EngPwr=global, FuelRate=global, LiftCmd=global
  wires:
  DOC/1(Out1) -> DPF/1(In1)
  DPF/1(Out1) -> SCR/1(In1)
  [Width] -> Statistics/2(Width[m])
  [VehSpd] -> Statistics/1(VehSpd [m/s])
  Statistics/3(Fuel [L]) -> Scope1/3  "Fuel[L]"
  [TravelDistance] -> Statistics/3(TravelDistance[m])
  Statistics/1(Distance [m]) -> Scope1/1  "Distance[m]"
  Statistics/2(Aera [ha]) -> Scope1/2  "Aera[ha]"
  [FuelRate] -> Statistics/4(FuelRate [mL/s])
  Statistics/5(LiftCmd [-]) -> [LiftCmd]
  Statistics/4(FuelRate [L/ha]) -> Scope1/4  "FuelRate[L/ha]"
  EngEmissionBus/1 -> DOC/1(EngInfo), Bus Selector/1
  Bus Selector/1 -> [FuelRate]  "<EngFuel[mL/s]>"
  Bus Selector/2 -> [EngPwr]  "<EngPwr[kW]>"
  [PwrPTO] -> Mux/2  "PwrPTO[kW]"
  Gain2/1 -> Scope2/1  "VehSpd[km/h]"
  [FuelRate] -> Gain/1
  Gain/1 -> Scope2/2  "FuelRate [L/h]"
  [PwrDraught] -> Mux/1  "PwrDraught[kW]"
  Mux/1 -> Scope2/3
  [VehSpd] -> Gain2/1  "VehSpd[m/s]"
  [EngPwr] -> Mux/3  "EngPwr [kW]"

== system Tractor_HIT_Discrete/DieselEngineModel ==
  EngSpd [rpm] : Inport
  Engine : Subsystem
  Engine1 : Subsystem  Commented=on
  Unit Delay : UnitDelay  SampleTime=-1  HasFrameUpgradeWarning=on
  EngTrq [Nm] : Outport
  EngEmissionBus : Outport  Port=2
  wires:
  Engine/1(EngTrq [Nm]) -> EngTrq [Nm]/1
  [LiftCmd] -> Engine/3(LiftCmd [-])
  [ThrottleCmd] -> Engine/2(ThrottleCmd [-])
  EngSpd [rpm]/1 -> Unit Delay/1
  Engine/2(EngInfo) -> EngEmissionBus/1
  Unit Delay/1 -> Engine/1(EngSpd [rpm])

== system Tractor_HIT_Discrete/ECU ==
  note: 改成%单位了
  EngineSpd_rpm : Inport
  ThrottleCmd_pct : Inport  Port=2
  EngineInfo : Inport  Port=3
  Bus Creator : BusCreator  Inputs=6
  Bus Selector : BusSelector  OutputSignals=FuelCyle,EGRRatio,RailPrs_kpa,IntakeMass,ExhTemp_DOC_in,ExhTemp_DOC_out,ExhTemp_DPF_out,ExhTemp_SCR_out,ExhMassFlow,mNOx_SCR_in,mNOx_SCR_out,Soot_Load,DPF_DP,NH3_Store,O2_frac
  ECU : Subsystem
  Gain{,1..4} (5 alike) : Gain
  EngineCmd : Outport
  wires:
  Bus Selector/13 -> ECU/14(DPF_DP)  "<DPF_DP>"
  Bus Selector/1 -> ECU/2(FuleCyle_mg)  "<FuelCyle>"
  Bus Selector/14 -> Gain3/1  "<NH3_Store>"
  Bus Selector/9 -> ECU/10(ExhMassFlow)  "<ExhMassFlow>"
  Bus Selector/3 -> ECU/4(RailPrs_kpa)  "<RailPrs_kpa>"
  EngineInfo/1 -> Bus Selector/1
  Bus Selector/10 -> ECU/11(mNOx_SCR_in)  "<mNOx_SCR_in>"
  Bus Selector/11 -> Gain2/1  "<mNOx_SCR_out>"
  Bus Selector/12 -> ECU/13(DPF_SootLoad)  "<Soot_Load>"
  Bus Selector/15 -> Gain4/1  "<O2_frac>"
  Bus Selector/2 -> ECU/3(EGRRatio)  "<EGRRatio>"
  Bus Selector/5 -> Gain/1  "<ExhTemp_DOC_in>"
  Bus Selector/4 -> ECU/5(IntakeMass)  "<IntakeMass>"
  Bus Selector/6 -> ECU/7(ExhTemp_DOC_out)  "<ExhTemp_DOC_out>"
  Bus Selector/7 -> ECU/8(ExhTemp_DPF_out)  "<ExhTemp_DPF_out>"
  Bus Selector/8 -> Gain1/1  "<ExhTemp_SCR_out>"
  ECU/3(EGROpeningTgt_pct) -> Bus Creator/3  "EGROpeningTgt_pct"
  ECU/2(FuelCyleTgt_mg) -> Bus Creator/2  "FuelCyleTgt_mg"
  ECU/6(mUREA_target) -> Bus Creator/6  "mUREA_target"
  ECU/1(EngineSpdTgt_rpm) -> Bus Creator/1  "EngineSpdTgt_rpm"
  ECU/5(DPF_regen_req) -> Bus Creator/5  "DPF_regen_req"
  ECU/4(PostInj_Request) -> Bus Creator/4  "PostInj_Request"
  EngineSpd_rpm/1 -> ECU/1(EngineSpd_rpm)
  Bus Creator/1 -> EngineCmd/1
  ThrottleCmd_pct/1 -> ECU/17(ThrottleCmd_pct)
  Gain/1 -> ECU/6(ExhTemp_DOC_in)
  Gain1/1 -> ECU/9(ExhTemp_SCR_out)
  Gain2/1 -> ECU/12(mNOx_SCR_out)
  Gain3/1 -> ECU/15(NH3_Store)
  Gain4/1 -> ECU/16(O2_frac)

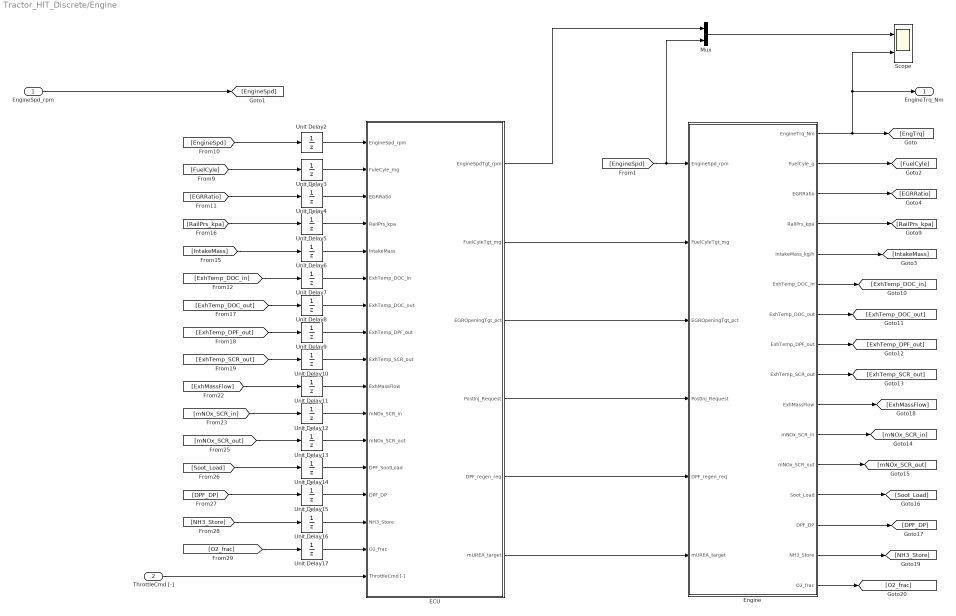
== system Tractor_HIT_Discrete/Engine ==
  EngineSpd_rpm : Inport
  ThrottleCmd [-] : Inport  Port=2
  ECU : Subsystem
  Engine : Subsystem
  Mux : Mux  Inputs=2
  Scope : Scope  NumInputPorts=2
  Unit Delay{2..17} (16 alike) : UnitDelay  SampleTime=-1  HasFrameUpgradeWarning=on
  EngineTrq_Nm : Outport
  wires:
  Engine/1(EngineTrq_Nm) -> [EngTrq], Scope/2, EngineTrq_Nm/1
  Engine/5(IntakeMass_kg/h) -> [IntakeMass]
  ECU/3(EGROpeningTgt_pct) -> Engine/3(EGROpeningTgt_pct)
  ECU/2(FuelCyleTgt_mg) -> Engine/2(FuelCyleTgt_mg)
  Engine/2(FuelCyle_g) -> [FuelCyle]
  ECU/5(DPF_regen_req) -> Engine/5(DPF_regen_req)
  ECU/6(mUREA_target) -> Engine/6(mUREA_target)
  Engine/3(EGRRatio) -> [EGRRatio]
  Engine/4(RailPrs_kpa) -> [RailPrs_kpa]
  Engine/6(ExhTemp_DOC_in) -> [ExhTemp_DOC_in]
  Engine/7(ExhTemp_DOC_out) -> [ExhTemp_DOC_out]
  Engine/9(ExhTemp_SCR_out) -> [ExhTemp_SCR_out]
  Engine/8(ExhTemp_DPF_out) -> [ExhTemp_DPF_out]
  Engine/13(Soot_Load) -> [Soot_Load]
  Engine/14(DPF_DP) -> [DPF_DP]
  Engine/12(mNOx_SCR_out) -> [mNOx_SCR_out]
  Engine/11(mNOx_SCR_in) -> [mNOx_SCR_in]
  Engine/10(ExhMassFlow) -> [ExhMassFlow]
  Engine/16(O2_frac) -> [O2_frac]
  Engine/15(NH3_Store) -> [NH3_Store]
  Unit Delay2/1 -> ECU/1(EngineSpd_rpm)
  [EngineSpd] -> Unit Delay2/1
  [FuelCyle] -> Unit Delay3/1
  Unit Delay3/1 -> ECU/2(FuleCyle_mg)
  Unit Delay5/1 -> ECU/4(RailPrs_kpa)
  [RailPrs_kpa] -> Unit Delay5/1
  [EGRRatio] -> Unit Delay4/1
  Unit Delay4/1 -> ECU/3(EGRRatio)
  Unit Delay8/1 -> ECU/7(ExhTemp_DOC_out)
  [ExhTemp_DOC_out] -> Unit Delay8/1
  [ExhTemp_DPF_out] -> Unit Delay9/1
  Unit Delay9/1 -> ECU/8(ExhTemp_DPF_out)
  Unit Delay7/1 -> ECU/6(ExhTemp_DOC_in)
  [ExhTemp_DOC_in] -> Unit Delay7/1
  [IntakeMass] -> Unit Delay6/1
  Unit Delay6/1 -> ECU/5(IntakeMass)
  Unit Delay14/1 -> ECU/13(DPF_SootLoad)
  [Soot_Load] -> Unit Delay14/1
  [DPF_DP] -> Unit Delay15/1
  Unit Delay15/1 -> ECU/14(DPF_DP)
  Unit Delay17/1 -> ECU/16(O2_frac)
  [O2_frac] -> Unit Delay17/1
  [NH3_Store] -> Unit Delay16/1
  Unit Delay16/1 -> ECU/15(NH3_Store)
  Unit Delay12/1 -> ECU/11(mNOx_SCR_in)
  [mNOx_SCR_in] -> Unit Delay12/1
  [mNOx_SCR_out] -> Unit Delay13/1
  Unit Delay13/1 -> ECU/12(mNOx_SCR_out)
  Unit Delay11/1 -> ECU/10(ExhMassFlow)
  [ExhMassFlow] -> Unit Delay11/1
  [ExhTemp_SCR_out] -> Unit Delay10/1
  Unit Delay10/1 -> ECU/9(ExhTemp_SCR_out)
  ThrottleCmd [-]/1 -> ECU/17(ThrottleCmd [-])
  ECU/4(PostInj_Request) -> Engine/4(PostInj_Request)
  [EngineSpd] -> Mux/2, Engine/1(EngineSpd_rpm)
  ECU/1(EngineSpdTgt_rpm) -> Mux/1
  Mux/1 -> Scope/1
  EngineSpd_rpm/1 -> [EngineSpd]

== system Tractor_HIT_Discrete/EngineModel ==
  EngineSpd_rpm : Inport
  EngineCmd : Inport  Port=2
  Bus Creator : BusCreator  Inputs=15
  Bus Selector : BusSelector  OutputSignals=FuelCyleTgt_mg,EGROpeningTgt_pct,PostInj_Request,DPF_regen_req,mUREA_target,EngineSpdTgt_rpm
  Engine1 : Subsystem
  Mux : Mux  Inputs=2
  Scope : Scope  NumInputPorts=2
  EngineTrq_Nm : Outport
  EngineInfo : Outport  Port=2
  wires:
  Engine1/10(ExhMassFlow) -> Bus Creator/9  "ExhMassFlow"
  Engine1/7(ExhTemp_DOC_out) -> Bus Creator/6  "ExhTemp_DOC_out"
  Engine1/13(Soot_Load) -> Bus Creator/12  "Soot_Load"
  Engine1/12(mNOx_SCR_out) -> Bus Creator/11  "mNOx_SCR_out"
  Engine1/5(IntakeMass_kg/h) -> Bus Creator/4  "IntakeMass"
  Engine1/4(RailPrs_kpa) -> Bus Creator/3  "RailPrs_kpa"
  Engine1/9(ExhTemp_SCR_out) -> Bus Creator/8  "ExhTemp_SCR_out"
  Engine1/8(ExhTemp_DPF_out) -> Bus Creator/7  "ExhTemp_DPF_out"
  Engine1/16(O2_frac) -> Bus Creator/15  "O2_frac"
  Engine1/11(mNOx_SCR_in) -> Bus Creator/10  "mNOx_SCR_in"
  Engine1/2(FuelCyle_mg) -> Bus Creator/1  "FuelCyle"
  Bus Creator/1 -> EngineInfo/1
  Engine1/15(NH3_Store) -> Bus Creator/14  "NH3_Store"
  Engine1/6(ExhTemp_DOC_in) -> Bus Creator/5  "ExhTemp_DOC_in"
  Engine1/3(EGRRatio) -> Bus Creator/2  "EGRRatio"
  Engine1/14(DPF_DP) -> Bus Creator/13  "DPF_DP"
  Engine1/1(EngineTrq_Nm) -> Scope/2, EngineTrq_Nm/1  "EngineTrq_Nm"
  EngineSpd_rpm/1 -> Mux/2, Engine1/1(EngineSpd_rpm)  "EngineSpd_rpm"
  EngineCmd/1 -> Bus Selector/1
  Bus Selector/3 -> Engine1/4(PostInj_Request)  "<PostInj_Request>"
  Bus Selector/4 -> Engine1/5(DPF_regen_req)  "<DPF_regen_req>"
  Bus Selector/2 -> Engine1/3(EGROpeningTgt_pct)  "<EGROpeningTgt_pct>"
  Bus Selector/5 -> Engine1/6(mUREA_target)  "<mUREA_target>"
  Bus Selector/1 -> Engine1/2(FuelCyleTgt_mg)  "<FuelCyleTgt_mg>"
  Bus Selector/6 -> [EngineSpdTgt_rpm]  "<EngineSpdTgt_rpm>"
  [EngineSpdTgt_rpm] -> Mux/1
  Mux/1 -> Scope/1

== system Tractor_HIT_Discrete/WorkloadModel ==
  EngTrq [Nm] : Inport
  Agricultural Implement : Subsystem
  Tires and Ground : Subsystem
  Tractor : Subsystem
  Transmission : Subsystem
  Unit Delay : UnitDelay  InitialCondition=0.01  SampleTime=-1  HasFrameUpgradeWarning=on
  Unit Delay1 : UnitDelay  InitialCondition=0.01  SampleTime=-1  HasFrameUpgradeWarning=on
  EngSpd [rpm] : Outport
  tag scope: PwrDraught=global, PwrPTO=global, VehSpd=global, Width=global
  wires:
  Tires and Ground/2(RollResis[N]) -> Tractor/2(RollRes[N])
  [GearCmd] -> Transmission/2(GearCmd[-])
  Transmission/3(AxlTrqR [Nm]) -> Tires and Ground/5(AxlTrqR [Nm])
  Tractor/1(VehSpd [m/s]) -> [VehSpd]
  Agricultural Implement/5(PwrDraught [kW]) -> [PwrDraught]
  Agricultural Implement/6(PwrPTO [kw]) -> [PwrPTO]
  Transmission/2(AxlTrqF [Nm]) -> Tires and Ground/4(AxlTrqF [Nm])
  [PTOSpdCmd] -> Agricultural Implement/2(PTOSpdCmd [-])
  Agricultural Implement/1(PTOTrq [Nm]) -> Transmission/4(PTOTrq [Nm])
  [Land] -> Agricultural Implement/6(Land [-])
  Tires and Ground/1(DriveForce[N]) -> Tractor/1(DriveForce[N])
  Transmission/1(EngSpd [rpm]) -> EngSpd [rpm]/1
  [Land] -> Tires and Ground/2(Land[-])
  [TypeCmd] -> Agricultural Implement/1(TypeCmd [-])
  [Scene] -> Tires and Ground/1(Scene[-])
  Tires and Ground/3(SlopeResis[N]) -> Tractor/3(SlopeResis[N])
  Agricultural Implement/3(TractiveResis [N]) -> Tractor/4(TractiveResis [N])
  EngTrq [Nm]/1 -> Transmission/3(EngTrq [Nm])
  [DriveCmd] -> Tires and Ground/3(DriveCmd [-]), Transmission/1(DriveCmd [-])
  Tires and Ground/4(WhlSpdR[m/s]) -> Transmission/6(WhlSpdR [m/s])
  [Scene] -> Agricultural Implement/5(Scene [-])
  Agricultural Implement/2(LiftTrq [Nm]) -> Transmission/5(LiftTrq [Nm])
  [VehSpd] -> Unit Delay1/1
  [VehSpd] -> Unit Delay/1
  Agricultural Implement/4(Width [m]) -> [Width]
  Unit Delay/1 -> Tires and Ground/6(VehSpd[m/s])
  [LiftCmd] -> Agricultural Implement/4(LiftCmd [-])
  Unit Delay1/1 -> Agricultural Implement/3(VehSpd [m/s])

== system Tractor_HIT_Discrete/DieselAftertreatmentSystem/DOC ==
  EngInfo : Inport
  Out1 : Outport
  wires:
  EngInfo/1 -> Out1/1

== system Tractor_HIT_Discrete/DieselAftertreatmentSystem/DPF ==
  In1 : Inport
  Out1 : Outport
  wires:
  In1/1 -> Out1/1

== system Tractor_HIT_Discrete/DieselAftertreatmentSystem/SCR ==
  In1 : Inport
  Bus Selector : BusSelector  OutputSignals=EngEoNOx[g/s],EngEoCO2[g/s],EngEoPM[g/s]
  Scope2 : Scope  NumInputPorts=3
  wires:
  In1/1 -> Bus Selector/1
  Bus Selector/1 -> Scope2/1  "<EngEoNOx[g/s]>"
  Bus Selector/2 -> Scope2/2  "<EngEoCO2[g/s]>"
  Bus Selector/3 -> Scope2/3  "<EngEoPM[g/s]>"

== system Tractor_HIT_Discrete/DieselAftertreatmentSystem/Statistics ==
  note: 1公顷=10000平方米
      | （hectare，ha）
  VehSpd [m/s] : Inport
  Width[m] : Inport  Port=2
  TravelDistance[m] : Inport  Port=3
  FuelRate [mL/s] : Inport  Port=4
  Discrete-Time Integrator : DiscreteIntegrator  SampleTime=-1  ICPrevOutput=DiscIntNeverNeededParam  ICPrevScaledInput=DiscIntNeverNeededParam
  Discrete-Time Integrator1 : DiscreteIntegrator  SampleTime=-1  ICPrevOutput=DiscIntNeverNeededParam  ICPrevScaledInput=DiscIntNeverNeededParam
  Discrete-Time Integrator2 : DiscreteIntegrator  SampleTime=-1  ICPrevOutput=DiscIntNeverNeededParam  ICPrevScaledInput=DiscIntNeverNeededParam
  Divide : Product  Inputs=*/
  Divide2 : Product  Inputs=*/
  Gain : Gain  Gain=0.95
  Gain1 : Gain  Gain=0.001
  GreaterThan : RelationalOperator  OutDataTypeStr=boolean  RndMeth=Simplest  InputSameDT=off
  Mod : Math  Operator=mod
  Product : Product
  Saturation : Saturate  UpperLimit=inf  LowerLimit=0.0001
  mm2ha : Constant  Value=1e4
  Distance [m] : Outport
  Aera [ha] : Outport  Port=2
  Fuel [L] : Outport  Port=3
  FuelRate [L/ha] : Outport  Port=4
  LiftCmd [-] : Outport  Port=5
  wires:
  Divide2/1 -> Discrete-Time Integrator1/1, Saturation/1
  mm2ha/1 -> Divide2/2
  Discrete-Time Integrator/1 -> Mod/1, Distance [m]/1  "Distance[m]"
  Discrete-Time Integrator1/1 -> Aera [ha]/1  "Aera[ha]"
  Gain/1 -> GreaterThan/2
  Discrete-Time Integrator2/1 -> Fuel [L]/1  "Fuel[L]"
  Gain1/1 -> Discrete-Time Integrator2/1, Divide/1
  Product/1 -> Divide2/1
  Saturation/1 -> Divide/2
  Divide/1 -> FuelRate [L/ha]/1  "FuelRate[L/ha]"
  VehSpd [m/s]/1 -> Discrete-Time Integrator/1, Product/1
  Mod/1 -> GreaterThan/1
  Width[m]/1 -> Product/2
  FuelRate [mL/s]/1 -> Gain1/1
  TravelDistance[m]/1 -> Gain/1, Mod/2
  GreaterThan/1 -> LiftCmd [-]/1  "LiftCmd[-]"
